simulink model "nms_sim_2D_cost"  (R2024b)
settings: Solver=ode15s  StartTime=0.0  StopTime=t_sim  MaxStep=dt_max  EnableMultiTasking=on
values from neighbouring files (symbols this model uses):
  a_BFSH = param_ctrl(35)*1    [setCtrlPar_optim_CPGreflex2001_2D.m]
  a_GAS = param_ctrl(37)*1    [setCtrlPar_optim_CPGreflex2001_2D.m]
  a_GLU = param_ctrl(31)*1    [setCtrlPar_optim_CPGreflex2001_2D.m]
  a_HAM = param_ctrl(33)*1    [setCtrlPar_optim_CPGreflex2001_2D.m]
  a_HFL = param_ctrl(32)*1    [setCtrlPar_optim_CPGreflex2001_2D.m]
  a_RF = param_ctrl(34)*1    [setCtrlPar_optim_CPGreflex2001_2D.m]
  a_SOL = param_ctrl(38)*1    [setCtrlPar_optim_CPGreflex2001_2D.m]
  a_TA = param_ctrl(39)*1    [setCtrlPar_optim_CPGreflex2001_2D.m]
  a_VAS = param_ctrl(36)*1    [setCtrlPar_optim_CPGreflex2001_2D.m]
  ai = param_ctrl(96)*2.0    [setCtrlPar_optim_CPGreflex2001_2D.m]
  b_BFSH = param_ctrl(52)*.51    [setCtrlPar_optim_CPGreflex2001_2D.m]
  b_BFSHGAS = param_ctrl(55)*.51    [setCtrlPar_optim_CPGreflex2001_2D.m]
  b_BFSHHAM = param_ctrl(54)*.51    [setCtrlPar_optim_CPGreflex2001_2D.m]
  b_BFSHVAS = param_ctrl(53)*.51    [setCtrlPar_optim_CPGreflex2001_2D.m]
  b_GAS = param_ctrl(59)*.51    [setCtrlPar_optim_CPGreflex2001_2D.m]
  b_GASBFSH = param_ctrl(60)*.51    [setCtrlPar_optim_CPGreflex2001_2D.m]
  b_GASSOL = param_ctrl(61)*.51    [setCtrlPar_optim_CPGreflex2001_2D.m]
  b_GLU = param_ctrl(40)*.51    [setCtrlPar_optim_CPGreflex2001_2D.m]
  b_GLUHAM = param_ctrl(42)*.51    [setCtrlPar_optim_CPGreflex2001_2D.m]
  b_GLUHFL = param_ctrl(41)*.51    [setCtrlPar_optim_CPGreflex2001_2D.m]
  b_HAM = param_ctrl(46)*.51    [setCtrlPar_optim_CPGreflex2001_2D.m]
  b_HAMBFSH = param_ctrl(48)*.51    [setCtrlPar_optim_CPGreflex2001_2D.m]
  b_HAMGLU = param_ctrl(47)*.51    [setCtrlPar_optim_CPGreflex2001_2D.m]
  b_HFL = param_ctrl(43)*.51    [setCtrlPar_optim_CPGreflex2001_2D.m]
  b_HFLGLU = param_ctrl(44)*.51    [setCtrlPar_optim_CPGreflex2001_2D.m]
  b_HFLRF = param_ctrl(45)*.51    [setCtrlPar_optim_CPGreflex2001_2D.m]
  b_RF = param_ctrl(49)*.51    [setCtrlPar_optim_CPGreflex2001_2D.m]
  b_RFHFL = param_ctrl(50)*.51    [setCtrlPar_optim_CPGreflex2001_2D.m]
  b_RFVAS = param_ctrl(51)*.51    [setCtrlPar_optim_CPGreflex2001_2D.m]
  b_SOL = param_ctrl(62)*.51    [setCtrlPar_optim_CPGreflex2001_2D.m]
  b_SOLGAS = param_ctrl(64)*.51    [setCtrlPar_optim_CPGreflex2001_2D.m]
  b_SOLTA = param_ctrl(63)*.51    [setCtrlPar_optim_CPGreflex2001_2D.m]
  b_TA = param_ctrl(65)*.51    [setCtrlPar_optim_CPGreflex2001_2D.m]
  b_TASOL = param_ctrl(66)*.51    [setCtrlPar_optim_CPGreflex2001_2D.m]
  b_VAS = param_ctrl(56)*.51    [setCtrlPar_optim_CPGreflex2001_2D.m]
  b_VASBFSH = param_ctrl(57)*.51    [setCtrlPar_optim_CPGreflex2001_2D.m]
  b_VASRF = param_ctrl(58)*.51    [setCtrlPar_optim_CPGreflex2001_2D.m]
  bias = param_ctrl(97)*2.5    [setCtrlPar_optim_CPGreflex2001_2D.m]
  c = 0.05    [nms_MS_2D_scaled.m]
  c_jointstop = 0.3 / (pi/180)    (= 17.1887338539)    [nms_MS_2D_scaled.m]
  D12_F = 0.16    *scaleL_JPhys    [nms_MechInit_2D_scaleSkel.m]
  D12_S = 0.2460	*sub_height    [nms_MechInit_2D_scaleSkel.m]
  D12_T = 0.2450  *sub_height    [nms_MechInit_2D_scaleSkel.m]
  D12y_F = 0.039  *sub_height    [nms_MechInit_2D_scaleSkel.m]
  D12z_HAT = 0.1    [nms_MS_2D_scaled.m]
  D13_F = 0.20    *scaleL_JPhys    [nms_MechInit_2D_scaleSkel.m]
  D1G_F = 0.14    *scaleL_JPhys    [nms_MechInit_2D_scaleSkel.m]
  D1G_HAT = 0.35  *scaleL_JPhys    [nms_MechInit_2D_scaleSkel.m]
  D1G_S = (0.3 - D12y_F/4)	*scaleL_JPhys    [nms_MechInit_2D_scaleSkel.m]
  D1G_T = (0.3 - D12y_F/4)	*scaleL_JPhys    [nms_MechInit_2D_scaleSkel.m]
  D1Gy_F = D12y_F*D1G_F/D12_F    (= 0.07)    [nms_MechInit_2D_scaleSkel.m]
  d_BFSH = param_ctrl(26)*1    [setCtrlPar_optim_CPGreflex2001_2D.m]
  d_GAS = param_ctrl(28)*1    [setCtrlPar_optim_CPGreflex2001_2D.m]
  d_GLU = param_ctrl(22)*1    [setCtrlPar_optim_CPGreflex2001_2D.m]
  d_HAM = param_ctrl(24)*1    [setCtrlPar_optim_CPGreflex2001_2D.m]
  d_HFL = param_ctrl(23)*1    [setCtrlPar_optim_CPGreflex2001_2D.m]
  d_RF = param_ctrl(25)*1    [setCtrlPar_optim_CPGreflex2001_2D.m]
  d_SOL = param_ctrl(29)*1    [setCtrlPar_optim_CPGreflex2001_2D.m]
  d_TA = param_ctrl(30)*1    [setCtrlPar_optim_CPGreflex2001_2D.m]
  d_VAS = param_ctrl(27)*1    [setCtrlPar_optim_CPGreflex2001_2D.m]
  DeltaThRef = 5e-3    (= 0.005)    [nms_MS_2D_scaled.m]
  dloptBFSH = 3.0    (= 3)    [setCtrlPar_optim_CPGreflex2001_2D.m]
  dloptGAS = 3.0    (= 3)    [setCtrlPar_optim_CPGreflex2001_2D.m]
  dloptGLU = 3.0    (= 3)    [setCtrlPar_optim_CPGreflex2001_2D.m]
  dloptHAM = 3.0    (= 3)    [setCtrlPar_optim_CPGreflex2001_2D.m]
  dloptHFL = 3.0    (= 3)    [setCtrlPar_optim_CPGreflex2001_2D.m]
  dloptRF = 3.0    (= 3)    [setCtrlPar_optim_CPGreflex2001_2D.m]
  dloptSOL = 3.0    (= 3)    [setCtrlPar_optim_CPGreflex2001_2D.m]
  dloptTA = 3.0    (= 3)    [setCtrlPar_optim_CPGreflex2001_2D.m]
  dloptVAS = 3.0    (= 3)    [setCtrlPar_optim_CPGreflex2001_2D.m]
  ec_BFSH = param_ctrl(80)*0.15    [setCtrlPar_optim_CPGreflex2001_2D.m]
  ec_GAS = param_ctrl(82)*0.15    [setCtrlPar_optim_CPGreflex2001_2D.m]
  ec_GLU = param_ctrl(76)*0.15    [setCtrlPar_optim_CPGreflex2001_2D.m]
  ec_HAM = param_ctrl(78)*0.15    [setCtrlPar_optim_CPGreflex2001_2D.m]
  ec_HFL = param_ctrl(77)*0.15    [setCtrlPar_optim_CPGreflex2001_2D.m]
  ec_RF = param_ctrl(79)*0.15    [setCtrlPar_optim_CPGreflex2001_2D.m]
  ec_TA = param_ctrl(84)*0.15    [setCtrlPar_optim_CPGreflex2001_2D.m]
  ec_VAS = param_ctrl(81)*0.15    [setCtrlPar_optim_CPGreflex2001_2D.m]
  eref = 0.04    [nms_MS_2D_scaled.m]
  eref_GAS = 0.1    [nms_MS_2D_scaled.m]
  eref_SOL = 0.1    [nms_MS_2D_scaled.m]
  es_BFSH = param_ctrl(89)*0.15    [setCtrlPar_optim_CPGreflex2001_2D.m]
  es_GAS = param_ctrl(91)*0.15    [setCtrlPar_optim_CPGreflex2001_2D.m]
  es_GLU = param_ctrl(85)*0.15    [setCtrlPar_optim_CPGreflex2001_2D.m]
  es_HAM = param_ctrl(87)*0.15    [setCtrlPar_optim_CPGreflex2001_2D.m]
  es_HFL = param_ctrl(86)*0.15    [setCtrlPar_optim_CPGreflex2001_2D.m]
  es_RF = param_ctrl(88)*0.15    [setCtrlPar_optim_CPGreflex2001_2D.m]
  es_TA = param_ctrl(93)*0.15    [setCtrlPar_optim_CPGreflex2001_2D.m]
  es_VAS = param_ctrl(90)*0.15    [setCtrlPar_optim_CPGreflex2001_2D.m]
  FmaxBFSH = 350    [nms_MS_2D_scaled.m]
  FmaxGAS = 2000    [nms_MS_2D_scaled.m]
  FmaxGLU = 4000    [nms_MS_2D_scaled.m]
  FmaxHAM = 2000    [nms_MS_2D_scaled.m]
  FmaxHFL = 2000    [nms_MS_2D_scaled.m]
  FmaxRF = 850    [nms_MS_2D_scaled.m]
  FmaxSOL = 4000    [nms_MS_2D_scaled.m]
  FmaxTA = 800    [nms_MS_2D_scaled.m]
  FmaxVAS = 5000    [nms_MS_2D_scaled.m]
  g = 9.81    [nms_MS_2D_scaled.m]
  gamma_4 = param_ctrl(11) * 1.7    [setCtrlPar_optim_CPGreflexsynergy2023_2D.m]
  h_BFSH = param_ctrl(71)*.1    [setCtrlPar_optim_CPGreflex2001_2D.m]
  h_GAS = param_ctrl(73)*.1    [setCtrlPar_optim_CPGreflex2001_2D.m]
  h_GLU = param_ctrl(67)*.1    [setCtrlPar_optim_CPGreflex2001_2D.m]
  h_HAM = param_ctrl(69)*.1    [setCtrlPar_optim_CPGreflex2001_2D.m]
  h_HFL = param_ctrl(68)*.1    [setCtrlPar_optim_CPGreflex2001_2D.m]
  h_RF = param_ctrl(70)*.1    [setCtrlPar_optim_CPGreflex2001_2D.m]
  h_SOL = param_ctrl(74)*.1    [setCtrlPar_optim_CPGreflex2001_2D.m]
  h_TA = param_ctrl(75)*.1    [setCtrlPar_optim_CPGreflex2001_2D.m]
  h_VAS = param_ctrl(72)*.1    [setCtrlPar_optim_CPGreflex2001_2D.m]
  HLCtrlPar = [theta_tgt l_clr alpha_tgt alpha_cd alpha_cv]    [setCtrlPar_optim_reflex2015_2D.m]
  In_F = 0.005    *scaleM*scaleL_JPhys^2    [nms_MechInit_2D_scaleSkel.m]
  In_HAT = 2.5    *scaleM*scaleL_JPhys^2    [nms_MechInit_2D_scaleSkel.m]
  In_S = 0.05     *scaleM*scaleL_JPhys^2    [nms_MechInit_2D_scaleSkel.m]
  In_T = 0.15     *scaleM*scaleL_JPhys^2    [nms_MechInit_2D_scaleSkel.m]
  init_exc = 0.01    [setInitPar_optim_2D.m]
  init_fm = 0.01    [setInitPar_optim_2D.m]
  init_lce = 1    [setInitPar_optim_2D.m]
  init_LCPG = param_ctrl(12) * 0.01    [setCtrlPar_optim_CPGreflexsynergy2023_2D.m]
  init_LStance = 1    [setInitPar_optim_2D.m]
  init_N1 = osc_signal1(phi_off_osc_ind)    [setCtrlPar_optim_CPGreflex2001_2D.m]
  ... (+441 more)
undefined symbols (not defined in the file or in its folder): cost_act_exponent, cost_v_tgt, flag_controller, Newton, nStep_obj, nStep_startKin, Raphson, sgn, SSW_kin, terrain_slope_angle, v_plateS1, X, Y, Z
libraries: nesl_utility x94, sm_lib x90, simulink x28, simulink_extras x12
(part 6 of 20)

== system nms_sim_2D_cost/Body Mechanics/cnt ==
  Cnt : Inport
  Cos : Trigonometry  Operator=cos
  Gain : Gain  Gain=-1
  Interpolation Using Prelookup : Interpolation_n-D  NumberOfTableDimensions=1  Table=v_plateZ  InternalRulePriority=Speed
      settings: InputPortMap=u0,u1
  Interpolation Using Prelookup1 : Interpolation_n-D  NumberOfTableDimensions=1  Table=v_plateS1  InterpMethod=Flat  InternalRulePriority=Speed
      settings: InputPortMap=u0,u1
  Mux : Mux  Inputs=5
  Prelookup : PreLookup  BreakpointsData=v_plateX  ExtrapMethod=Linear
  Selector : Selector  InputPortWidth=2  IndexOptions=Index vector (dialog)  Indices=1  OutputSizes=1
  Sin : Trigonometry
  Env : Outport
  wires:
  Cnt/1 -> Selector/1
  Prelookup/1 -> Interpolation Using Prelookup1/1, Interpolation Using Prelookup/1
  Prelookup/2 -> Interpolation Using Prelookup1/2, Interpolation Using Prelookup/2
  Selector/1 -> Prelookup/1, Mux/2
  Interpolation Using Prelookup/1 -> Mux/3, Mux/1
  Interpolation Using Prelookup1/1 -> Sin/1, Cos/1
  Sin/1 -> Gain/1
  Cos/1 -> Mux/5
  Gain/1 -> Mux/4
  Mux/1 -> Env/1

== system nms_sim_2D_cost/Body Mechanics/cnt1 ==
  Cnt : Inport
  Cos : Trigonometry  Operator=cos
  Gain : Gain  Gain=-1
  Interpolation Using Prelookup : Interpolation_n-D  NumberOfTableDimensions=1  Table=v_plateZ  InternalRulePriority=Speed
      settings: InputPortMap=u0,u1
  Interpolation Using Prelookup1 : Interpolation_n-D  NumberOfTableDimensions=1  Table=v_plateS1  InterpMethod=Flat  InternalRulePriority=Speed
      settings: InputPortMap=u0,u1
  Mux : Mux  Inputs=5
  Prelookup : PreLookup  BreakpointsData=v_plateX  ExtrapMethod=Linear
  Selector : Selector  InputPortWidth=2  IndexOptions=Index vector (dialog)  Indices=1  OutputSizes=1
  Sin : Trigonometry
  Env : Outport
  wires:
  Mux/1 -> Env/1
  Gain/1 -> Mux/4
  Cos/1 -> Mux/5
  Sin/1 -> Gain/1
  Interpolation Using Prelookup1/1 -> Cos/1, Sin/1
  Interpolation Using Prelookup/1 -> Mux/1, Mux/3
  Selector/1 -> Mux/2, Prelookup/1
  Prelookup/2 -> Interpolation Using Prelookup/2, Interpolation Using Prelookup1/2
  Prelookup/1 -> Interpolation Using Prelookup/1, Interpolation Using Prelookup1/1
  Cnt/1 -> Selector/1

== system nms_sim_2D_cost/Body Mechanics/cnt2 ==
  Cnt : Inport
  Cos : Trigonometry  Operator=cos
  Gain : Gain  Gain=-1
  Interpolation Using Prelookup : Interpolation_n-D  NumberOfTableDimensions=1  Table=v_plateZ  InternalRulePriority=Speed
      settings: InputPortMap=u0,u1
  Interpolation Using Prelookup1 : Interpolation_n-D  NumberOfTableDimensions=1  Table=v_plateS1  InterpMethod=Flat  InternalRulePriority=Speed
      settings: InputPortMap=u0,u1
  Mux : Mux  Inputs=5
  Prelookup : PreLookup  BreakpointsData=v_plateX  ExtrapMethod=Linear
  Selector : Selector  InputPortWidth=2  IndexOptions=Index vector (dialog)  Indices=1  OutputSizes=1
  Sin : Trigonometry
  Env : Outport
  wires:
  Cnt/1 -> Selector/1
  Prelookup/1 -> Interpolation Using Prelookup1/1, Interpolation Using Prelookup/1
  Prelookup/2 -> Interpolation Using Prelookup1/2, Interpolation Using Prelookup/2
  Selector/1 -> Prelookup/1, Mux/2
  Interpolation Using Prelookup/1 -> Mux/3, Mux/1
  Interpolation Using Prelookup1/1 -> Sin/1, Cos/1
  Sin/1 -> Gain/1
  Cos/1 -> Mux/5
  Gain/1 -> Mux/4
  Mux/1 -> Env/1

== system nms_sim_2D_cost/Body Mechanics/cnt3 ==
  Cnt : Inport
  Cos : Trigonometry  Operator=cos
  Gain : Gain  Gain=-1
  Interpolation Using Prelookup : Interpolation_n-D  NumberOfTableDimensions=1  Table=v_plateZ  InternalRulePriority=Speed
      settings: InputPortMap=u0,u1
  Interpolation Using Prelookup1 : Interpolation_n-D  NumberOfTableDimensions=1  Table=v_plateS1  InterpMethod=Flat  InternalRulePriority=Speed
      settings: InputPortMap=u0,u1
  Mux : Mux  Inputs=5
  Prelookup : PreLookup  BreakpointsData=v_plateX  ExtrapMethod=Linear
  Selector : Selector  InputPortWidth=2  IndexOptions=Index vector (dialog)  Indices=1  OutputSizes=1
  Sin : Trigonometry
  Env : Outport
  wires:
  Mux/1 -> Env/1
  Gain/1 -> Mux/4
  Cos/1 -> Mux/5
  Sin/1 -> Gain/1
  Interpolation Using Prelookup1/1 -> Cos/1, Sin/1
  Interpolation Using Prelookup/1 -> Mux/1, Mux/3
  Selector/1 -> Mux/2, Prelookup/1
  Prelookup/2 -> Interpolation Using Prelookup/2, Interpolation Using Prelookup1/2
  Prelookup/1 -> Interpolation Using Prelookup/1, Interpolation Using Prelookup1/1
  Cnt/1 -> Selector/1

== system nms_sim_2D_cost/Body Mechanics/contact information ==
  point : Inport
  Constant : Constant  Value=0
  Constant1 : Constant  Value=[0 0 1]
  Mux9 : Mux  Inputs=3
  Selector13 : Selector  InputPortWidth=3  IndexOptions=Index vector (dialog)  Indices=1  OutputSizes=1
  vector : Outport
  wires:
  Constant/1 -> Mux9/1
  Constant1/1 -> Mux9/3
  Mux9/1 -> vector/1
  point/1 -> Selector13/1
  Selector13/1 -> Mux9/2

== system nms_sim_2D_cost/Body Mechanics/contact information1 ==
  point : Inport
  Constant : Constant  Value=0
  Constant1 : Constant  Value=[0 0 1]
  Mux9 : Mux  Inputs=3
  Selector13 : Selector  InputPortWidth=3  IndexOptions=Index vector (dialog)  Indices=1  OutputSizes=1
  vector : Outport
  wires:
  Constant/1 -> Mux9/1
  Constant1/1 -> Mux9/3
  Mux9/1 -> vector/1
  point/1 -> Selector13/1
  Selector13/1 -> Mux9/2

== system nms_sim_2D_cost/Body Mechanics/contact information2 ==
  point : Inport
  Constant : Constant  Value=0
  Constant1 : Constant  Value=[0 0 1]
  Mux9 : Mux  Inputs=3
  Selector13 : Selector  InputPortWidth=3  IndexOptions=Index vector (dialog)  Indices=1  OutputSizes=1
  vector : Outport
  wires:
  Constant/1 -> Mux9/1
  Constant1/1 -> Mux9/3
  Mux9/1 -> vector/1
  point/1 -> Selector13/1
  Selector13/1 -> Mux9/2

== system nms_sim_2D_cost/Body Mechanics/contact information3 ==
  point : Inport
  Constant : Constant  Value=0
  Constant1 : Constant  Value=[0 0 1]
  Mux9 : Mux  Inputs=3
  Selector13 : Selector  InputPortWidth=3  IndexOptions=Index vector (dialog)  Indices=1  OutputSizes=1
  vector : Outport
  wires:
  Constant/1 -> Mux9/1
  Constant1/1 -> Mux9/3
  Mux9/1 -> vector/1
  point/1 -> Selector13/1
  Selector13/1 -> Mux9/2

== system nms_sim_2D_cost/CPG-reflex Controller/Alpha moto-neuron ==
  rhythm_ext : Inport
  GGLU : Inport  Port=2
  LMSHFL : Inport  Port=3
  LMSHAM : Inport  Port=4
  SGLU : Inport  Port=5
  Feedback : Inport  Port=6
  Constant : Constant  Value=h_GLU
  Gain1 : Gain  Gain=a_GLU
  Gain2 : Gain  Gain=1/tao_alpha
  Gain3 : Gain  Gain=d_GLU
  Gain4 : Gain  Gain=b_GLU
  Gain5 : Gain  Gain=-b_GLUHFL
  Gain6 : Gain  Gain=b_GLUHAM
  Gain7 : Gain  Gain=-1
  Integrator : Integrator  InitialCondition=init_exc
  Sum : Sum  Inputs=++++++++
  sigmoid function : Subsystem
  LExcGLU : Outport
  wires:
  Sum/1 -> Gain2/1, sigmoid function/1(u)
  SGLU/1 -> Gain4/1
  GGLU/1 -> Gain1/1
  rhythm_ext/1 -> Gain3/1
  Gain2/1 -> Integrator/1
  Integrator/1 -> Gain7/1
  Gain3/1 -> Sum/2
  Gain1/1 -> Sum/3
  Gain4/1 -> Sum/4
  Constant/1 -> Sum/8
  Feedback/1 -> Sum/7
  LMSHAM/1 -> Gain6/1
  LMSHFL/1 -> Gain5/1
  Gain5/1 -> Sum/5
  Gain6/1 -> Sum/6
  sigmoid function/1(LExcGLU) -> LExcGLU/1
  Gain7/1 -> Sum/1

== system nms_sim_2D_cost/CPG-reflex Controller/Alpha moto-neuron1 ==
  rhythm_ext : Inport
  GHAM : Inport  Port=2
  LMSGLU : Inport  Port=3
  LMSBFSH : Inport  Port=4
  SHAM : Inport  Port=5
  FBHAM : Inport  Port=6
  Constant : Constant  Value=h_HAM
  Gain1 : Gain  Gain=a_HAM
  Gain2 : Gain  Gain=1/tao_alpha
  Gain3 : Gain  Gain=d_HAM
  Gain4 : Gain  Gain=b_HAM
  Gain5 : Gain  Gain=b_HAMGLU
  Gain6 : Gain  Gain=b_HAMBFSH
  Gain7 : Gain  Gain=-1
  Integrator : Integrator  InitialCondition=init_exc
  Sum : Sum  Inputs=++++++++
  sigmoid function : Subsystem
  LExcHAM : Outport
  wires:
  Sum/1 -> Gain2/1, sigmoid function/1(u)
  SHAM/1 -> Gain4/1
  GHAM/1 -> Gain1/1
  rhythm_ext/1 -> Gain3/1
  Gain2/1 -> Integrator/1
  Integrator/1 -> Gain7/1
  Gain3/1 -> Sum/2
  Gain1/1 -> Sum/3
  Gain4/1 -> Sum/4
  Constant/1 -> Sum/8
  FBHAM/1 -> Sum/7
  LMSBFSH/1 -> Gain6/1
  LMSGLU/1 -> Gain5/1
  Gain5/1 -> Sum/5
  Gain6/1 -> Sum/6
  sigmoid function/1(LExcHAM) -> LExcHAM/1
  Gain7/1 -> Sum/1

== system nms_sim_2D_cost/CPG-reflex Controller/Alpha moto-neuron18 ==
  rhythm_ext : Inport
  GHAM : Inport  Port=2
  LMSGLU : Inport  Port=3
  LMSBFSH : Inport  Port=4
  SHAM : Inport  Port=5
  FBHAM : Inport  Port=6
  Constant : Constant  Value=h_HAM
  Gain1 : Gain  Gain=a_HAM
  Gain2 : Gain  Gain=1/tao_alpha
  Gain3 : Gain  Gain=d_HAM
  Gain4 : Gain  Gain=b_HAM
  Gain5 : Gain  Gain=b_HAMGLU
  Gain6 : Gain  Gain=b_HAMBFSH
  Gain7 : Gain  Gain=-1
  Integrator : Integrator  InitialCondition=init_exc
  Sum : Sum  Inputs=++++++++
  sigmoid function : Subsystem
  RExcHAM : Outport
  wires:
  Gain6/1 -> Sum/6
  Gain5/1 -> Sum/5
  LMSGLU/1 -> Gain5/1
  LMSBFSH/1 -> Gain6/1
  FBHAM/1 -> Sum/7
  Constant/1 -> Sum/8
  Gain4/1 -> Sum/4
  Gain1/1 -> Sum/3
  Gain3/1 -> Sum/2
  Integrator/1 -> Gain7/1
  Gain2/1 -> Integrator/1
  rhythm_ext/1 -> Gain3/1
  GHAM/1 -> Gain1/1
  SHAM/1 -> Gain4/1
  sigmoid function/1(RExc) -> RExcHAM/1
  Sum/1 -> sigmoid function/1(u), Gain2/1
  Gain7/1 -> Sum/1

== system nms_sim_2D_cost/CPG-reflex Controller/Alpha moto-neuron19 ==
  rhythm_flex : Inport
  GHFL : Inport  Port=2
  LMSGLU : Inport  Port=3
  LMSRF : Inport  Port=4
  SHFL : Inport  Port=5
  FBHFL : Inport  Port=6
  Constant : Constant  Value=h_HFL
  Gain1 : Gain  Gain=a_HFL
  Gain2 : Gain  Gain=1/tao_alpha
  Gain3 : Gain  Gain=d_HFL
  Gain4 : Gain  Gain=b_HFL
  Gain5 : Gain  Gain=-b_HFLGLU
  Gain6 : Gain  Gain=b_HFLRF
  Gain7 : Gain  Gain=-1
  Integrator : Integrator  InitialCondition=init_exc
  Scope1 : Scope
  Sum : Sum  Inputs=++++++++
  sigmoid function : Subsystem
  RExcHFL : Outport
  wires:
  Gain6/1 -> Sum/6
  Gain5/1 -> Sum/5
  LMSGLU/1 -> Gain5/1
  LMSRF/1 -> Gain6/1
  FBHFL/1 -> Sum/7
  Constant/1 -> Sum/8
  SHFL/1 -> Gain4/1
  GHFL/1 -> Gain1/1
  rhythm_flex/1 -> Gain3/1
  Gain2/1 -> Integrator/1
  Integrator/1 -> Gain7/1
  Gain3/1 -> Sum/2
  Gain1/1 -> Sum/3
  Gain4/1 -> Sum/4
  Sum/1 -> sigmoid function/1(u), Gain2/1
  sigmoid function/1(RExc) -> RExcHFL/1
  Gain7/1 -> Sum/1, Scope1/1

== system nms_sim_2D_cost/CPG-reflex Controller/Alpha moto-neuron2 ==
  rhythm_flex : Inport
  GHFL : Inport  Port=2
  LMSGLU : Inport  Port=3
  LMSRF : Inport  Port=4
  SHFL : Inport  Port=5
  FBHFL : Inport  Port=6
  Constant : Constant  Value=h_HFL
  Gain1 : Gain  Gain=a_HFL
  Gain2 : Gain  Gain=tao_alpha
  Gain3 : Gain  Gain=d_HFL
  Gain4 : Gain  Gain=b_HFL
  Gain5 : Gain  Gain=-b_HFLGLU
  Gain6 : Gain  Gain=b_HFLRF
  Gain7 : Gain  Gain=-1
  Integrator : Integrator  InitialCondition=1
  Sum : Sum  Inputs=++++++++
  sigmoid function : Subsystem
  LExcHFL : Outport
  wires:
  Gain4/1 -> Sum/4
  Gain1/1 -> Sum/3
  Gain3/1 -> Sum/2
  Integrator/1 -> Gain7/1
  Gain2/1 -> Integrator/1
  rhythm_flex/1 -> Gain3/1
  GHFL/1 -> Gain1/1
  SHFL/1 -> Gain4/1
  Constant/1 -> Sum/8
  FBHFL/1 -> Sum/7
  LMSRF/1 -> Gain6/1
  LMSGLU/1 -> Gain5/1
  Gain5/1 -> Sum/5
  Gain6/1 -> Sum/6
  Sum/1 -> sigmoid function/1(u), Gain2/1
  sigmoid function/1(LExc) -> LExcHFL/1
  Gain7/1 -> Sum/1

== system nms_sim_2D_cost/CPG-reflex Controller/Alpha moto-neuron20 ==
  rhythm_flex : Inport
  GRF : Inport  Port=2
  LMSHFL : Inport  Port=3
  LMSVAS : Inport  Port=4
  SRF : Inport  Port=5
  FBRF : Inport  Port=6
  Constant : Constant  Value=h_RF
  Gain1 : Gain  Gain=a_RF
  Gain2 : Gain  Gain=1/tao_alpha
  Gain3 : Gain  Gain=d_RF
  Gain4 : Gain  Gain=b_RF
  Gain5 : Gain  Gain=b_RFHFL
  Gain6 : Gain  Gain=b_RFVAS
  Gain7 : Gain  Gain=-1
  Integrator : Integrator  InitialCondition=init_exc
  Sum : Sum  Inputs=++++++++
  sigmoid function : Subsystem
  RExcRF : Outport
  wires:
  Gain6/1 -> Sum/6
  LMSVAS/1 -> Gain6/1
  Gain5/1 -> Sum/5
  LMSHFL/1 -> Gain5/1
  FBRF/1 -> Sum/7
  Constant/1 -> Sum/8
  SRF/1 -> Gain4/1
  GRF/1 -> Gain1/1
  rhythm_flex/1 -> Gain3/1
  Gain2/1 -> Integrator/1
  Integrator/1 -> Gain7/1
  Gain3/1 -> Sum/2
  Gain1/1 -> Sum/3
  Gain4/1 -> Sum/4
  sigmoid function/1(RExc) -> RExcRF/1
  Sum/1 -> sigmoid function/1(u), Gain2/1
  Gain7/1 -> Sum/1

== system nms_sim_2D_cost/CPG-reflex Controller/Alpha moto-neuron21 ==
  rhythm_ext : Inport
  GBFSH : Inport  Port=2
  LMSVAS : Inport  Port=3
  LMSGAS : Inport  Port=4
  LMSHAM : Inport  Port=5
  SBFSH : Inport  Port=6
  FBBFSH : Inport  Port=7
  Constant : Constant  Value=h_BFSH
  Gain1 : Gain  Gain=a_BFSH
  Gain2 : Gain  Gain=1/tao_alpha
  Gain3 : Gain  Gain=d_BFSH
  Gain4 : Gain  Gain=b_BFSH
  Gain5 : Gain  Gain=-b_BFSHVAS
  Gain6 : Gain  Gain=b_BFSHGAS
  Gain7 : Gain  Gain=b_BFSHHAM
  Gain8 : Gain  Gain=-1
  Integrator : Integrator  InitialCondition=init_exc
  Sum : Sum  Inputs=+++++++++
  sigmoid function : Subsystem
  RExcBFSH : Outport
  wires:
  Gain7/1 -> Sum/7
  Gain6/1 -> Sum/6
  Gain5/1 -> Sum/5
  LMSVAS/1 -> Gain5/1
  LMSGAS/1 -> Gain6/1
  LMSHAM/1 -> Gain7/1
  FBBFSH/1 -> Sum/8
  Constant/1 -> Sum/9
  SBFSH/1 -> Gain4/1
  GBFSH/1 -> Gain1/1
  rhythm_ext/1 -> Gain3/1
  Gain2/1 -> Integrator/1
  Integrator/1 -> Gain8/1
  Gain3/1 -> Sum/2
  Gain1/1 -> Sum/3
  Gain4/1 -> Sum/4
  Sum/1 -> sigmoid function/1(u), Gain2/1
  sigmoid function/1(RExc) -> RExcBFSH/1
  Gain8/1 -> Sum/1

== system nms_sim_2D_cost/CPG-reflex Controller/Alpha moto-neuron22 ==
  rhythm_flex : Inport
  GVAS : Inport  Port=2
  LMSBFSH : Inport  Port=3
  LMSRF : Inport  Port=4
  SVAS : Inport  Port=5
  FBVAS : Inport  Port=6
  Constant : Constant  Value=h_VAS
  Gain1 : Gain  Gain=a_VAS
  Gain2 : Gain  Gain=1/tao_alpha
  Gain3 : Gain  Gain=d_VAS
  Gain4 : Gain  Gain=b_VAS
  Gain5 : Gain  Gain=b_VASRF
  Gain6 : Gain  Gain=-b_VASBFSH
  Gain7 : Gain  Gain=-1
  Integrator : Integrator  InitialCondition=init_exc
  Sum : Sum  Inputs=++++++++
  sigmoid function : Subsystem
  RExcVAS : Outport
  wires:
  Gain6/1 -> Sum/5  "msbfsh"
  Gain5/1 -> Sum/6  "msrf"
  LMSRF/1 -> Gain5/1
  LMSBFSH/1 -> Gain6/1
  FBVAS/1 -> Sum/7  "fb"
  Constant/1 -> Sum/8  "h"
  Gain4/1 -> Sum/4  "ms"
  Gain1/1 -> Sum/3  "golgi"
  Gain3/1 -> Sum/2  "rhythm"
  Integrator/1 -> Gain7/1  "aloha"
  Gain2/1 -> Integrator/1
  rhythm_flex/1 -> Gain3/1
  GVAS/1 -> Gain1/1
  SVAS/1 -> Gain4/1
  Sum/1 -> sigmoid function/1(u), Gain2/1
  sigmoid function/1(RExc) -> RExcVAS/1
  Gain7/1 -> Sum/1

== system nms_sim_2D_cost/CPG-reflex Controller/Alpha moto-neuron23 ==
  rhythm_ext : Inport
  GSOL : Inport  Port=2
  LMSTA : Inport  Port=3
  LMSGAS : Inport  Port=4
  SSOL : Inport  Port=5
  FB SOL : Inport  Port=6
  Constant : Constant  Value=h_SOL
  Gain1 : Gain  Gain=a_SOL
  Gain2 : Gain  Gain=1/tao_alpha
  Gain3 : Gain  Gain=d_SOL
  Gain4 : Gain  Gain=b_SOL
  Gain5 : Gain  Gain=-b_SOLTA
  Gain6 : Gain  Gain=b_SOLGAS
  Gain7 : Gain  Gain=-1
  Integrator : Integrator  InitialCondition=init_exc
  Sum : Sum  Inputs=++++++++
  sigmoid function : Subsystem
  RExcSOL : Outport
  wires:
  Gain6/1 -> Sum/6
  Gain5/1 -> Sum/5
  LMSTA/1 -> Gain5/1
  LMSGAS/1 -> Gain6/1
  FB SOL/1 -> Sum/7
  Constant/1 -> Sum/8
  Gain4/1 -> Sum/4
  Gain1/1 -> Sum/3
  Gain3/1 -> Sum/2
  Integrator/1 -> Gain7/1
  Gain2/1 -> Integrator/1
  rhythm_ext/1 -> Gain3/1
  GSOL/1 -> Gain1/1
  SSOL/1 -> Gain4/1
  sigmoid function/1(RExc) -> RExcSOL/1
  Sum/1 -> sigmoid function/1(u), Gain2/1
  Gain7/1 -> Sum/1

== system nms_sim_2D_cost/CPG-reflex Controller/Alpha moto-neuron24 ==
  rhythm_flex : Inport
  GTA : Inport  Port=2
  LMSSOL : Inport  Port=3
  STA : Inport  Port=4
  FB TA : Inport  Port=5
  Constant : Constant  Value=h_TA
  Gain1 : Gain  Gain=a_TA
  Gain2 : Gain  Gain=1/tao_alpha
  Gain3 : Gain  Gain=d_TA
  Gain4 : Gain  Gain=b_TA
  Gain5 : Gain  Gain=-b_TASOL
  Gain7 : Gain  Gain=-1
  Integrator : Integrator  InitialCondition=init_exc
  Sum : Sum  Inputs=+++++++
  sigmoid function : Subsystem
  RExcTA : Outport
  wires:
  FB TA/1 -> Sum/6
  Gain5/1 -> Sum/5
  LMSSOL/1 -> Gain5/1
  Constant/1 -> Sum/7
  STA/1 -> Gain4/1
  GTA/1 -> Gain1/1
  rhythm_flex/1 -> Gain3/1
  Gain2/1 -> Integrator/1
  Integrator/1 -> Gain7/1
  Gain3/1 -> Sum/2
  Gain1/1 -> Sum/3
  Gain4/1 -> Sum/4
  Sum/1 -> sigmoid function/1(u), Gain2/1
  Gain7/1 -> Sum/1
  sigmoid function/1(RExc) -> RExcTA/1

== system nms_sim_2D_cost/CPG-reflex Controller/Alpha moto-neuron25 ==
  rhythm_ext : Inport
  GGAS : Inport  Port=2
  LMSBFSH : Inport  Port=3
  LMSSOL : Inport  Port=4
  SGAS : Inport  Port=5
  FBGAS : Inport  Port=6
  Constant : Constant  Value=h_GAS
  Gain1 : Gain  Gain=a_GAS
  Gain2 : Gain  Gain=1/tao_alpha
  Gain3 : Gain  Gain=d_GAS
  Gain4 : Gain  Gain=b_GAS
  Gain5 : Gain  Gain=b_GASBFSH
  Gain6 : Gain  Gain=b_GASSOL
  Gain7 : Gain  Gain=-1
  Integrator : Integrator  InitialCondition=init_exc
  Sum : Sum  Inputs=++++++++
  sigmoid function : Subsystem
  RExcGAS : Outport
  wires:
  Gain6/1 -> Sum/6
  Gain5/1 -> Sum/5
  LMSBFSH/1 -> Gain5/1
  LMSSOL/1 -> Gain6/1
  FBGAS/1 -> Sum/7
  Constant/1 -> Sum/8
  SGAS/1 -> Gain4/1
  GGAS/1 -> Gain1/1
  rhythm_ext/1 -> Gain3/1
  Gain2/1 -> Integrator/1
  Integrator/1 -> Gain7/1
  Gain3/1 -> Sum/2
  Gain1/1 -> Sum/3
  Gain4/1 -> Sum/4
  Sum/1 -> sigmoid function/1(u), Gain2/1
  sigmoid function/1(RExc) -> RExcGAS/1
  Gain7/1 -> Sum/1

== system nms_sim_2D_cost/CPG-reflex Controller/Alpha moto-neuron26 ==
  rhythm_ext : Inport
  GGLU : Inport  Port=2
  LMSHFL : Inport  Port=3
  LMSHAM : Inport  Port=4
  SGLU : Inport  Port=5
  Feedback : Inport  Port=6
  Constant : Constant  Value=h_GLU
  Gain1 : Gain  Gain=a_GLU
  Gain2 : Gain  Gain=1/tao_alpha
  Gain3 : Gain  Gain=d_GLU
  Gain4 : Gain  Gain=b_GLU
  Gain5 : Gain  Gain=-b_GLUHFL
  Gain6 : Gain  Gain=b_GLUHAM
  Gain7 : Gain  Gain=-1
  Integrator : Integrator  InitialCondition=init_exc
  Sum : Sum  Inputs=++++++++
  sigmoid function : Subsystem
  RExcGLU : Outport
  wires:
  Gain6/1 -> Sum/6
  Gain5/1 -> Sum/5
  LMSHFL/1 -> Gain5/1
  LMSHAM/1 -> Gain6/1
  Feedback/1 -> Sum/7
  Constant/1 -> Sum/8
  Gain4/1 -> Sum/4
  Gain1/1 -> Sum/3
  Gain3/1 -> Sum/2
  Integrator/1 -> Gain7/1
  Gain2/1 -> Integrator/1
  rhythm_ext/1 -> Gain3/1
  GGLU/1 -> Gain1/1
  SGLU/1 -> Gain4/1
  sigmoid function/1(RExc) -> RExcGLU/1
  Sum/1 -> Gain2/1, sigmoid function/1(u)
  Gain7/1 -> Sum/1

== system nms_sim_2D_cost/CPG-reflex Controller/Alpha moto-neuron3 ==
  rhythm_flex : Inport
  GRF : Inport  Port=2
  LMSHFL : Inport  Port=3
  LMSVAS : Inport  Port=4
  SRF : Inport  Port=5
  FBRF : Inport  Port=6
  Constant : Constant  Value=h_RF
  Gain1 : Gain  Gain=a_RF
  Gain2 : Gain  Gain=1/tao_alpha
  Gain3 : Gain  Gain=d_RF
  Gain4 : Gain  Gain=b_RF
  Gain5 : Gain  Gain=b_RFHFL
  Gain6 : Gain  Gain=b_RFVAS
  Gain7 : Gain  Gain=-1
  Integrator : Integrator  InitialCondition=init_exc
  Sum : Sum  Inputs=++++++++
  sigmoid function : Subsystem
  LExcRF : Outport
  wires:
  Gain4/1 -> Sum/4
  Gain1/1 -> Sum/3
  Gain3/1 -> Sum/2
  Integrator/1 -> Gain7/1
  Gain2/1 -> Integrator/1
  rhythm_flex/1 -> Gain3/1
  GRF/1 -> Gain1/1
  SRF/1 -> Gain4/1
  Constant/1 -> Sum/8
  FBRF/1 -> Sum/7
  LMSHFL/1 -> Gain5/1
  Gain5/1 -> Sum/5
  LMSVAS/1 -> Gain6/1
  Gain6/1 -> Sum/6
  Sum/1 -> sigmoid function/1(u), Gain2/1
  sigmoid function/1(LExc) -> LExcRF/1
  Gain7/1 -> Sum/1

== system nms_sim_2D_cost/CPG-reflex Controller/Alpha moto-neuron4 ==
  rhythm_ext : Inport
  GBFSH : Inport  Port=2
  LMSVAS : Inport  Port=3
  LMSGAS : Inport  Port=4
  LMSHAM : Inport  Port=5
  SBFSH : Inport  Port=6
  FBBFSH : Inport  Port=7
  Constant : Constant  Value=h_BFSH
  Gain1 : Gain  Gain=a_BFSH
  Gain2 : Gain  Gain=1/tao_alpha
  Gain3 : Gain  Gain=d_BFSH
  Gain4 : Gain  Gain=b_BFSH
  Gain5 : Gain  Gain=-b_BFSHVAS
  Gain6 : Gain  Gain=b_BFSHGAS
  Gain7 : Gain  Gain=b_BFSHHAM
  Gain8 : Gain  Gain=-1
  Integrator : Integrator  InitialCondition=init_exc
  Sum : Sum  Inputs=+++++++++
  sigmoid function : Subsystem
  LExcBFSH : Outport
  wires:
  Gain4/1 -> Sum/4
  Gain1/1 -> Sum/3
  Gain3/1 -> Sum/2
  Integrator/1 -> Gain8/1
  Gain2/1 -> Integrator/1
  rhythm_ext/1 -> Gain3/1
  GBFSH/1 -> Gain1/1
  SBFSH/1 -> Gain4/1
  Constant/1 -> Sum/9
  FBBFSH/1 -> Sum/8
  LMSHAM/1 -> Gain7/1
  LMSGAS/1 -> Gain6/1
  LMSVAS/1 -> Gain5/1
  Gain5/1 -> Sum/5
  Gain6/1 -> Sum/6
  Gain7/1 -> Sum/7
  Sum/1 -> sigmoid function/1(u), Gain2/1
  sigmoid function/1(LExcBFSH) -> LExcBFSH/1
  Gain8/1 -> Sum/1

== system nms_sim_2D_cost/CPG-reflex Controller/Alpha moto-neuron5 ==
  rhythm_flex : Inport
  GVAS : Inport  Port=2
  LMSBFSH : Inport  Port=3
  LMSRF : Inport  Port=4
  SVAS : Inport  Port=5
  FBVAS : Inport  Port=6
  Constant : Constant  Value=h_VAS
  Gain1 : Gain  Gain=a_VAS
  Gain2 : Gain  Gain=1/tao_alpha
  Gain3 : Gain  Gain=d_VAS
  Gain4 : Gain  Gain=b_VAS
  Gain5 : Gain  Gain=b_VASRF
  Gain6 : Gain  Gain=-b_VASBFSH
  Gain7 : Gain  Gain=-1
  Integrator : Integrator  InitialCondition=init_exc
  Sum : Sum  Inputs=++++++++
  sigmoid function : Subsystem
  LExcVAS : Outport
  wires:
  SVAS/1 -> Gain4/1
  GVAS/1 -> Gain1/1
  rhythm_flex/1 -> Gain3/1
  Gain2/1 -> Integrator/1
  Integrator/1 -> Gain7/1
  Gain3/1 -> Sum/2
  Gain1/1 -> Sum/3
  Gain4/1 -> Sum/4
  Constant/1 -> Sum/8
  FBVAS/1 -> Sum/7
  LMSBFSH/1 -> Gain6/1
  LMSRF/1 -> Gain5/1
  Gain5/1 -> Sum/6
  Gain6/1 -> Sum/5
  Sum/1 -> sigmoid function/1(u), Gain2/1
  Gain7/1 -> Sum/1
  sigmoid function/1(LExc) -> LExcVAS/1

== system nms_sim_2D_cost/CPG-reflex Controller/Alpha moto-neuron6 ==
  rhythm_ext : Inport
  GSOL : Inport  Port=2
  LMSTA : Inport  Port=3
  LMSGAS : Inport  Port=4
  SSOL : Inport  Port=5
  FB SOL : Inport  Port=6
  Constant : Constant  Value=h_SOL
  Gain1 : Gain  Gain=a_SOL
  Gain2 : Gain  Gain=1/tao_alpha
  Gain3 : Gain  Gain=d_SOL
  Gain4 : Gain  Gain=b_SOL
  Gain5 : Gain  Gain=-b_SOLTA
  Gain6 : Gain  Gain=b_SOLGAS
  Gain7 : Gain  Gain=-1
  Integrator : Integrator  InitialCondition=init_exc
  Sum : Sum  Inputs=++++++++
  sigmoid function : Subsystem
  LExcSOL : Outport
  wires:
  SSOL/1 -> Gain4/1
  GSOL/1 -> Gain1/1
  rhythm_ext/1 -> Gain3/1
  Gain2/1 -> Integrator/1
  Integrator/1 -> Gain7/1  "alpha"
  Gain3/1 -> Sum/2  "rhythm"
  Gain1/1 -> Sum/3  "golgi"
  Gain4/1 -> Sum/4  "ms"
  Constant/1 -> Sum/8  "h"
  FB SOL/1 -> Sum/7  "fb"
  LMSGAS/1 -> Gain6/1
  LMSTA/1 -> Gain5/1
  Gain5/1 -> Sum/5  "msta"
  Gain6/1 -> Sum/6  "msgas"
  sigmoid function/1(LExcSOL) -> LExcSOL/1
  Sum/1 -> sigmoid function/1(u), Gain2/1
  Gain7/1 -> Sum/1

== system nms_sim_2D_cost/CPG-reflex Controller/Alpha moto-neuron7 ==
  rhythm_flex : Inport
  GTA : Inport  Port=2
  LMSSOL : Inport  Port=3
  STA : Inport  Port=4
  FB TA : Inport  Port=5
  Constant : Constant  Value=h_TA
  Gain1 : Gain  Gain=a_TA
  Gain2 : Gain  Gain=1/tao_alpha
  Gain3 : Gain  Gain=d_TA
  Gain4 : Gain  Gain=b_TA
  Gain5 : Gain  Gain=-b_TASOL
  Gain7 : Gain  Gain=-1
  Integrator : Integrator  InitialCondition=init_exc
  Sum : Sum  Inputs=+++++++
  sigmoid function : Subsystem
  LExcTA : Outport
  wires:
  Gain4/1 -> Sum/4
  Gain1/1 -> Sum/3
  Gain3/1 -> Sum/2
  Integrator/1 -> Gain7/1
  Gain2/1 -> Integrator/1
  rhythm_flex/1 -> Gain3/1
  GTA/1 -> Gain1/1
  STA/1 -> Gain4/1
  Constant/1 -> Sum/7
  LMSSOL/1 -> Gain5/1
  Gain5/1 -> Sum/5
  FB TA/1 -> Sum/6
  sigmoid function/1(LExcTA) -> LExcTA/1
  Sum/1 -> sigmoid function/1(u), Gain2/1
  Gain7/1 -> Sum/1

== system nms_sim_2D_cost/CPG-reflex Controller/Alpha moto-neuron8 ==
  rhythm_ext : Inport
  GGAS : Inport  Port=2
  LMSBFSH : Inport  Port=3
  LMSSOL : Inport  Port=4
  SGAS : Inport  Port=5
  FBGAS : Inport  Port=6
  Constant : Constant  Value=h_GAS
  Gain1 : Gain  Gain=a_GAS
  Gain2 : Gain  Gain=1/tao_alpha
  Gain3 : Gain  Gain=d_GAS
  Gain4 : Gain  Gain=b_GAS
  Gain5 : Gain  Gain=b_GASBFSH
  Gain6 : Gain  Gain=b_GASSOL
  Gain7 : Gain  Gain=-1
  Integrator : Integrator  InitialCondition=init_exc
  Sum : Sum  Inputs=++++++++
  sigmoid function : Subsystem
  LExcGAS : Outport
  wires:
  Gain4/1 -> Sum/4
  Gain1/1 -> Sum/3
  Gain3/1 -> Sum/2
  Integrator/1 -> Gain7/1
  Gain2/1 -> Integrator/1
  rhythm_ext/1 -> Gain3/1
  GGAS/1 -> Gain1/1
  SGAS/1 -> Gain4/1
  Constant/1 -> Sum/8
  FBGAS/1 -> Sum/7
  LMSSOL/1 -> Gain6/1
  LMSBFSH/1 -> Gain5/1
  Gain5/1 -> Sum/5
  Gain6/1 -> Sum/6
  sigmoid function/1(LExcBFSH) -> LExcGAS/1
  Sum/1 -> sigmoid function/1(u), Gain2/1
  Gain7/1 -> Sum/1

== system nms_sim_2D_cost/CPG-reflex Controller/CPG ==
  note: Adaptation
  note: Adaptation
  note: External stimulation
  note: Neuron 1
  note: Neuron 2
  FB : Inport
  Constant5 : Constant  Value=s_ext
  Gain1 : Gain  Gain=1/tao_r
  Gain10 : Gain  Gain=-1
  Gain11 : Gain  Gain=1/tao_a
  Gain14 : Gain  Gain=-1
  Gain15 : Gain  Gain=1/tao_a
  Gain16 : Gain  Gain=ai
  Gain17 : Gain  Gain=bias
  Gain18 : Gain  Gain=ai
  Gain2 : Gain  Gain=bias
  Gain3 : Gain  Gain=1/tao_r
  Integrator4 : Integrator  InitialCondition=init_N1
  Integrator5 : Integrator  InitialCondition=init_V1
  Integrator6 : Integrator  InitialCondition=init_N2
  Integrator7 : Integrator  InitialCondition=init_V2
  Max2 : MinMax  Function=max  Inputs=2
  Max3 : MinMax  Function=max  Inputs=2
  Sum4 : Sum  Inputs=--+-+
  Sum5 : Sum
  Sum6 : Sum  Inputs=--+-+
  Sum7 : Sum
  Zero : Constant  Value=0  OutDataTypeStr=Inherit: Inherit via back propagation
  Zero1 : Constant  Value=0  OutDataTypeStr=Inherit: Inherit via back propagation
  Outport : Outport
  Outport1 : Outport  Port=2
  wires:
  FB/1 -> Sum6/5, Sum4/5
  Sum5/1 -> Gain11/1
  Gain3/1 -> Integrator6/1
  Zero1/1 -> Max3/2
  Constant5/1 -> [s]
  Gain11/1 -> Integrator5/1
  Gain16/1 -> Sum6/4  "-a*max(x2, 0)"
  Zero/1 -> Max2/2
  Gain18/1 -> Sum4/4  "-a*max(x2, 0)"
  Integrator4/1 -> Max2/1, Sum4/1  "x"
  Max2/1 -> Sum5/2, Gain16/1, Outport/1
  Sum6/1 -> Gain3/1
  Gain10/1 -> Sum5/1  "-f"
  Sum4/1 -> Gain1/1
  Gain14/1 -> Sum7/1  "-f"
  Integrator7/1 -> Gain17/1, Gain14/1  "f"
  Integrator6/1 -> Sum6/1, Max3/1  "x"
  Max3/1 -> Sum7/2, Outport1/1, Gain18/1
  Gain2/1 -> Sum4/2  "bf"
  Gain1/1 -> Integrator4/1
  [s] -> Sum6/3  "s"
  Gain17/1 -> Sum6/2  "bf"
  [s] -> Sum4/3  "s"
  Gain15/1 -> Integrator7/1
  Sum7/1 -> Gain15/1
  Integrator5/1 -> Gain10/1, Gain2/1  "f"

== system nms_sim_2D_cost/CPG-reflex Controller/FB VAS ==
  LStance : Inport
  Constant : Constant
  Gain : Gain  Gain=ec_VAS
  Gain1 : Gain  Gain=es_VAS
  Sum : Sum  Inputs=|-+
  Sum1 : Sum  Inputs=|++
  FBVAS : Outport
  wires:
  LStance/1 -> Sum/1, Gain/1
  Constant/1 -> Sum/2
  Gain/1 -> Sum1/1
  Sum1/1 -> FBVAS/1
  Sum/1 -> Gain1/1
  Gain1/1 -> Sum1/2

== system nms_sim_2D_cost/CPG-reflex Controller/FB VAS2 ==
  RStance : Inport
  Constant : Constant
  Gain : Gain  Gain=ec_VAS
  Gain1 : Gain  Gain=es_VAS
  Sum : Sum  Inputs=|-+
  Sum1 : Sum  Inputs=|++
  FBVAS : Outport
  wires:
  Gain1/1 -> Sum1/2
  Sum/1 -> Gain1/1
  Sum1/1 -> FBVAS/1
  Gain/1 -> Sum1/1
  Constant/1 -> Sum/2
  RStance/1 -> Gain/1, Sum/1

== system nms_sim_2D_cost/CPG-reflex Controller/Feedback HAM ==
  LStance : Inport
  Constant : Constant
  Gain : Gain  Gain=ec_HAM
  Gain1 : Gain  Gain=es_HAM
  Sum : Sum  Inputs=|-+
  Sum1 : Sum  Inputs=|++
  FBHAM : Outport
  wires:
  LStance/1 -> Sum/1, Gain/1
  Constant/1 -> Sum/2
  Gain/1 -> Sum1/1
  Sum1/1 -> FBHAM/1
  Sum/1 -> Gain1/1
  Gain1/1 -> Sum1/2

== system nms_sim_2D_cost/CPG-reflex Controller/Feedback HAM2 ==
  RStance : Inport
  Constant : Constant
  Gain : Gain  Gain=ec_HAM
  Gain1 : Gain  Gain=es_HAM
  Sum : Sum  Inputs=|-+
  Sum1 : Sum  Inputs=|++
  FBHAM : Outport
  wires:
  Gain1/1 -> Sum1/2
  Sum/1 -> Gain1/1
  Sum1/1 -> FBHAM/1
  Gain/1 -> Sum1/1
  Constant/1 -> Sum/2
  RStance/1 -> Gain/1, Sum/1

== system nms_sim_2D_cost/CPG-reflex Controller/Golgi tendon organ BFSH ==
  FBFSH : Inport
  Gain : Gain  Gain=-1
  Gain1 : Gain  Gain=1/tao_golgi
  Integrator : Integrator  InitialCondition=init_fm
  Max : MinMax  Function=max  Inputs=2
  Sum : Sum
  Zero : Constant  Value=0  OutDataTypeStr=Inherit: Inherit via back propagation
  GBFSH : Outport
  wires:
  Gain1/1 -> Integrator/1
  Sum/1 -> Max/1, Gain1/1
  FBFSH/1 -> Sum/2
  Gain/1 -> Sum/1
  Integrator/1 -> Gain/1
  Zero/1 -> Max/2
  Max/1 -> GBFSH/1

== system nms_sim_2D_cost/CPG-reflex Controller/Golgi tendon organ BFSH2 ==
  FBFSH : Inport
  Gain : Gain  Gain=-1
  Gain1 : Gain  Gain=1/tao_golgi
  Integrator : Integrator  InitialCondition=init_fm
  Max : MinMax  Function=max  Inputs=2
  Sum : Sum
  Zero : Constant  Value=0  OutDataTypeStr=Inherit: Inherit via back propagation
  GBFSH : Outport
  wires:
  Max/1 -> GBFSH/1
  Zero/1 -> Max/2
  Integrator/1 -> Gain/1
  Gain/1 -> Sum/1
  FBFSH/1 -> Sum/2
  Sum/1 -> Gain1/1, Max/1
  Gain1/1 -> Integrator/1

== system nms_sim_2D_cost/CPG-reflex Controller/Golgi tendon organ GAS ==
  FmGAS : Inport
  Gain : Gain  Gain=-1
  Gain1 : Gain  Gain=1/tao_golgi
  Integrator : Integrator  InitialCondition=init_fm
  Max : MinMax  Function=max  Inputs=2
  Sum : Sum
  Zero : Constant  Value=0  OutDataTypeStr=Inherit: Inherit via back propagation
  GGAS : Outport
  wires:
  Gain1/1 -> Integrator/1
  Sum/1 -> Max/1, Gain1/1
  FmGAS/1 -> Sum/2
  Gain/1 -> Sum/1
  Integrator/1 -> Gain/1
  Zero/1 -> Max/2
  Max/1 -> GGAS/1

== system nms_sim_2D_cost/CPG-reflex Controller/Golgi tendon organ GAS2 ==
  FmGAS : Inport
  Gain : Gain  Gain=-1
  Gain1 : Gain  Gain=1/tao_golgi
  Integrator : Integrator  InitialCondition=init_fm
  Max : MinMax  Function=max  Inputs=2
  Sum : Sum
  Zero : Constant  Value=0  OutDataTypeStr=Inherit: Inherit via back propagation
  GGAS : Outport
  wires:
  Max/1 -> GGAS/1
  Zero/1 -> Max/2
  Integrator/1 -> Gain/1
  Gain/1 -> Sum/1
  FmGAS/1 -> Sum/2
  Sum/1 -> Gain1/1, Max/1
  Gain1/1 -> Integrator/1

== system nms_sim_2D_cost/CPG-reflex Controller/Golgi tendon organ GLU ==
  Fm : Inport
  Gain : Gain  Gain=-1
  Gain1 : Gain  Gain=1/tao_golgi
  Integrator : Integrator  InitialCondition=init_fm
  Max : MinMax  Function=max  Inputs=2
  Sum : Sum
  Zero : Constant  Value=0  OutDataTypeStr=Inherit: Inherit via back propagation
  Gm : Outport
  wires:
  Max/1 -> Gm/1
  Zero/1 -> Max/2
  Integrator/1 -> Gain/1
  Gain/1 -> Sum/1
  Fm/1 -> Sum/2
  Sum/1 -> Gain1/1, Max/1
  Gain1/1 -> Integrator/1

== system nms_sim_2D_cost/CPG-reflex Controller/Golgi tendon organ GLU2 ==
  Fm : Inport
  Gain : Gain  Gain=-1
  Gain1 : Gain  Gain=1/tao_golgi
  Integrator : Integrator  InitialCondition=init_fm
  Max : MinMax  Function=max  Inputs=2
  Sum : Sum
  Zero : Constant  Value=0  OutDataTypeStr=Inherit: Inherit via back propagation
  GGLU : Outport
  wires:
  Gain1/1 -> Integrator/1
  Sum/1 -> Max/1, Gain1/1
  Fm/1 -> Sum/2
  Gain/1 -> Sum/1
  Integrator/1 -> Gain/1
  Zero/1 -> Max/2
  Max/1 -> GGLU/1

== system nms_sim_2D_cost/CPG-reflex Controller/Golgi tendon organ HAM ==
  Fm : Inport
  Gain : Gain  Gain=-1
  Gain1 : Gain  Gain=1/tao_golgi
  Integrator : Integrator  InitialCondition=init_fm
  Max : MinMax  Function=max  Inputs=2
  Sum : Sum
  Zero : Constant  Value=0  OutDataTypeStr=Inherit: Inherit via back propagation
  Gm : Outport
  wires:
  Max/1 -> Gm/1
  Zero/1 -> Max/2
  Integrator/1 -> Gain/1
  Gain/1 -> Sum/1
  Fm/1 -> Sum/2
  Sum/1 -> Gain1/1, Max/1
  Gain1/1 -> Integrator/1

== system nms_sim_2D_cost/CPG-reflex Controller/Golgi tendon organ HAM2 ==
  FHAM : Inport
  Gain : Gain  Gain=-1
  Gain1 : Gain  Gain=1/tao_golgi
  Integrator : Integrator  InitialCondition=init_fm
  Max : MinMax  Function=max  Inputs=2
  Sum : Sum
  Zero : Constant  Value=0  OutDataTypeStr=Inherit: Inherit via back propagation
  GHAM : Outport
  wires:
  Gain1/1 -> Integrator/1
  Sum/1 -> Max/1, Gain1/1
  FHAM/1 -> Sum/2
  Gain/1 -> Sum/1
  Integrator/1 -> Gain/1
  Zero/1 -> Max/2
  Max/1 -> GHAM/1

== system nms_sim_2D_cost/CPG-reflex Controller/Golgi tendon organ HFL ==
  FmHFL : Inport
  Gain : Gain  Gain=-1
  Gain1 : Gain  Gain=1/tao_golgi
  Integrator : Integrator  InitialCondition=init_fm
  Max : MinMax  Function=max  Inputs=2
  Sum : Sum
  Zero : Constant  Value=0  OutDataTypeStr=Inherit: Inherit via back propagation
  GHFL : Outport
  wires:
  Gain1/1 -> Integrator/1
  Sum/1 -> Max/1, Gain1/1
  FmHFL/1 -> Sum/2
  Gain/1 -> Sum/1
  Integrator/1 -> Gain/1
  Zero/1 -> Max/2
  Max/1 -> GHFL/1

== system nms_sim_2D_cost/CPG-reflex Controller/Golgi tendon organ HFL2 ==
  FmHFL : Inport
  Gain : Gain  Gain=-1
  Gain1 : Gain  Gain=1/tao_golgi
  Integrator : Integrator  InitialCondition=init_fm
  Max : MinMax  Function=max  Inputs=2
  Sum : Sum
  Zero : Constant  Value=0  OutDataTypeStr=Inherit: Inherit via back propagation
  GHFL : Outport
  wires:
  Max/1 -> GHFL/1
  Zero/1 -> Max/2
  Integrator/1 -> Gain/1
  Gain/1 -> Sum/1
  FmHFL/1 -> Sum/2
  Sum/1 -> Gain1/1, Max/1
  Gain1/1 -> Integrator/1

== system nms_sim_2D_cost/CPG-reflex Controller/Golgi tendon organ RF ==
  FRF : Inport
  Gain : Gain  Gain=-1
  Gain1 : Gain  Gain=1/tao_golgi
  Integrator : Integrator  InitialCondition=init_fm
  Max : MinMax  Function=max  Inputs=2
  Sum : Sum
  Zero : Constant  Value=0  OutDataTypeStr=Inherit: Inherit via back propagation
  GRF : Outport
  wires:
  Gain1/1 -> Integrator/1
  Sum/1 -> Max/1, Gain1/1
  FRF/1 -> Sum/2
  Gain/1 -> Sum/1
  Integrator/1 -> Gain/1
  Zero/1 -> Max/2
  Max/1 -> GRF/1

== system nms_sim_2D_cost/CPG-reflex Controller/Golgi tendon organ RF2 ==
  FRF : Inport
  Gain : Gain  Gain=-1
  Gain1 : Gain  Gain=1/tao_golgi
  Integrator : Integrator  InitialCondition=init_fm
  Max : MinMax  Function=max  Inputs=2
  Sum : Sum
  Zero : Constant  Value=0  OutDataTypeStr=Inherit: Inherit via back propagation
  GRF : Outport
  wires:
  Max/1 -> GRF/1
  Zero/1 -> Max/2
  Integrator/1 -> Gain/1
  Gain/1 -> Sum/1
  FRF/1 -> Sum/2
  Sum/1 -> Gain1/1, Max/1
  Gain1/1 -> Integrator/1

== system nms_sim_2D_cost/CPG-reflex Controller/Golgi tendon organ SOL ==
  FmSOL : Inport
  Gain : Gain  Gain=-1
  Gain1 : Gain  Gain=1/tao_golgi
  Integrator : Integrator  InitialCondition=init_fm
  Max : MinMax  Function=max  Inputs=2
  Sum : Sum
  Zero : Constant  Value=0  OutDataTypeStr=Inherit: Inherit via back propagation
  GSOL : Outport
  wires:
  Max/1 -> GSOL/1
  Zero/1 -> Max/2
  Integrator/1 -> Gain/1
  Gain/1 -> Sum/1
  FmSOL/1 -> Sum/2
  Sum/1 -> Gain1/1, Max/1
  Gain1/1 -> Integrator/1

== system nms_sim_2D_cost/CPG-reflex Controller/Golgi tendon organ SOL2 ==
  FmSOL : Inport
  Gain : Gain  Gain=-1
  Gain1 : Gain  Gain=1/tao_golgi
  Integrator : Integrator  InitialCondition=init_fm
  Max : MinMax  Function=max  Inputs=2
  Sum : Sum
  Zero : Constant  Value=0  OutDataTypeStr=Inherit: Inherit via back propagation
  GSOL : Outport
  wires:
  Gain1/1 -> Integrator/1
  Sum/1 -> Max/1, Gain1/1
  FmSOL/1 -> Sum/2
  Gain/1 -> Sum/1
  Integrator/1 -> Gain/1
  Zero/1 -> Max/2
  Max/1 -> GSOL/1

== system nms_sim_2D_cost/CPG-reflex Controller/Golgi tendon organ TA ==
  FTA : Inport
  Gain : Gain  Gain=-1
  Gain1 : Gain  Gain=1/tao_golgi
  Integrator : Integrator  InitialCondition=init_fm
  Max : MinMax  Function=max  Inputs=2
  Sum : Sum
  Zero : Constant  Value=0  OutDataTypeStr=Inherit: Inherit via back propagation
  GTA : Outport
  wires:
  Gain1/1 -> Integrator/1
  Sum/1 -> Max/1, Gain1/1
  FTA/1 -> Sum/2
  Gain/1 -> Sum/1
  Integrator/1 -> Gain/1
  Zero/1 -> Max/2
  Max/1 -> GTA/1

== system nms_sim_2D_cost/CPG-reflex Controller/Golgi tendon organ TA2 ==
  FTA : Inport
  Gain : Gain  Gain=-1
  Gain1 : Gain  Gain=1/tao_golgi
  Integrator : Integrator  InitialCondition=init_fm
  Max : MinMax  Function=max  Inputs=2
  Sum : Sum
  Zero : Constant  Value=0  OutDataTypeStr=Inherit: Inherit via back propagation
  GTA : Outport
  wires:
  Max/1 -> GTA/1
  Zero/1 -> Max/2
  Integrator/1 -> Gain/1
  Gain/1 -> Sum/1
  FTA/1 -> Sum/2
  Sum/1 -> Gain1/1, Max/1
  Gain1/1 -> Integrator/1

== system nms_sim_2D_cost/CPG-reflex Controller/Golgi tendon organ VAS ==
  FmVAS : Inport
  Gain : Gain  Gain=-1
  Gain1 : Gain  Gain=1/tao_golgi
  Integrator : Integrator  InitialCondition=init_fm
  Max : MinMax  Function=max  Inputs=2
  Sum : Sum
  Zero : Constant  Value=0  OutDataTypeStr=Inherit: Inherit via back propagation
  GVAS : Outport
  wires:
  Max/1 -> GVAS/1
  Zero/1 -> Max/2
  Integrator/1 -> Gain/1
  Gain/1 -> Sum/1
  FmVAS/1 -> Sum/2
  Sum/1 -> Gain1/1, Max/1
  Gain1/1 -> Integrator/1

== system nms_sim_2D_cost/CPG-reflex Controller/Golgi tendon organ VAS2 ==
  FmVAS : Inport
  Gain : Gain  Gain=-1
  Gain1 : Gain  Gain=1/tao_golgi
  Integrator : Integrator  InitialCondition=init_fm
  Max : MinMax  Function=max  Inputs=2
  Sum : Sum
  Zero : Constant  Value=0  OutDataTypeStr=Inherit: Inherit via back propagation
  GVAS : Outport
  wires:
  Gain1/1 -> Integrator/1
  Sum/1 -> Max/1, Gain1/1
  FmVAS/1 -> Sum/2
  Gain/1 -> Sum/1
  Integrator/1 -> Gain/1
  Zero/1 -> Max/2
  Max/1 -> GVAS/1

== system nms_sim_2D_cost/CPG-reflex Controller/Muscle Spindle BFSH ==
  note: Lm
  Lce : Inport
  Vce : Inport  Port=2
  Constant2 : Constant
  Constant3 : Constant  Value=0
  Constant4 : Constant
  Gain2 : Gain  Gain=1/tao_spindle
  Gain3 : Gain  Gain=p_BFSH
  Gain4 : Gain  Gain=q_BFSH
  GreaterThan : RelationalOperator  OutDataTypeStr=boolean  RndMeth=Simplest  InputSameDT=off
  Integrator : Integrator  InitialCondition=init_lce
  Saturation : Saturate  UpperLimit=inf  LowerLimit=0
  Saturation1 : Saturate  UpperLimit=inf  LowerLimit=0
  Saturation2 : Saturate  UpperLimit=inf  LowerLimit=0
  Sum4 : Sum  Inputs=|+-
  Sum5 : Sum  Inputs=-++
  Switch : Switch  Criteria=u2 > Threshold  SaturateOnIntegerOverflow=off  InputSameDT=off
  Sm : Outport
  wires:
  Constant2/1 -> Sum4/2
  Saturation/1 -> Gain4/1
  Constant3/1 -> Switch/3
  Constant4/1 -> GreaterThan/2
  GreaterThan/1 -> Switch/2
  Switch/1 -> Sm/1  "Sm"
  Saturation2/1 -> Switch/1
  Gain2/1 -> Integrator/1
  Lce/1 -> Sum4/1, GreaterThan/1  "Lm"
  Saturation1/1 -> Gain3/1
  Gain4/1 -> Sum5/2
  Sum5/1 -> Saturation2/1, Gain2/1
  Integrator/1 -> Sum5/1
  Gain3/1 -> Sum5/3
  Sum4/1 -> Saturation/1
  Vce/1 -> Saturation1/1  "vm"

== system nms_sim_2D_cost/CPG-reflex Controller/Muscle Spindle BFSH2 ==
  note: Lm
  Lce : Inport
  Vce : Inport  Port=2
  Constant2 : Constant
  Constant3 : Constant  Value=0
  Constant4 : Constant
  Gain2 : Gain  Gain=1/tao_spindle
  Gain3 : Gain  Gain=p_BFSH
  Gain4 : Gain  Gain=q_BFSH
  GreaterThan : RelationalOperator  OutDataTypeStr=boolean  RndMeth=Simplest  InputSameDT=off
  Integrator : Integrator  InitialCondition=init_lce
  Saturation : Saturate  UpperLimit=inf  LowerLimit=0
  Saturation1 : Saturate  UpperLimit=inf  LowerLimit=0
  Saturation2 : Saturate  UpperLimit=inf  LowerLimit=0
  Sum4 : Sum  Inputs=|+-
  Sum5 : Sum  Inputs=-++
  Switch : Switch  Criteria=u2 > Threshold  SaturateOnIntegerOverflow=off  InputSameDT=off
  Sm : Outport
  wires:
  Constant2/1 -> Sum4/2
  Saturation/1 -> Gain4/1
  Constant3/1 -> Switch/3
  Constant4/1 -> GreaterThan/2
  GreaterThan/1 -> Switch/2
  Switch/1 -> Sm/1  "Sm"
  Saturation2/1 -> Switch/1
  Gain2/1 -> Integrator/1
  Lce/1 -> Sum4/1, GreaterThan/1  "Lm"
  Saturation1/1 -> Gain3/1
  Gain4/1 -> Sum5/2
  Sum5/1 -> Saturation2/1, Gain2/1
  Integrator/1 -> Sum5/1
  Gain3/1 -> Sum5/3
  Sum4/1 -> Saturation/1
  Vce/1 -> Saturation1/1  "vm"

== system nms_sim_2D_cost/CPG-reflex Controller/Muscle Spindle GAS ==
  note: Lm
  Lce : Inport
  Vce : Inport  Port=2
  Constant2 : Constant
  Constant3 : Constant  Value=0
  Constant4 : Constant
  Gain2 : Gain  Gain=1/tao_spindle
  Gain3 : Gain  Gain=p_GAS
  Gain4 : Gain  Gain=q_GAS
  GreaterThan : RelationalOperator  OutDataTypeStr=boolean  RndMeth=Simplest  InputSameDT=off
  Integrator : Integrator  InitialCondition=init_lce
  Saturation : Saturate  UpperLimit=inf  LowerLimit=0
  Saturation1 : Saturate  UpperLimit=inf  LowerLimit=0
  Saturation2 : Saturate  UpperLimit=inf  LowerLimit=0
  Sum4 : Sum  Inputs=|+-
  Sum5 : Sum  Inputs=-++
  Switch : Switch  Criteria=u2 > Threshold  SaturateOnIntegerOverflow=off  InputSameDT=off
  Sm : Outport
  wires:
  Constant2/1 -> Sum4/2
  Saturation/1 -> Gain4/1
  Constant3/1 -> Switch/3
  Constant4/1 -> GreaterThan/2
  GreaterThan/1 -> Switch/2
  Switch/1 -> Sm/1  "Sm"
  Saturation2/1 -> Switch/1
  Gain2/1 -> Integrator/1
  Lce/1 -> Sum4/1, GreaterThan/1  "Lm"
  Saturation1/1 -> Gain3/1
  Gain4/1 -> Sum5/2
  Sum5/1 -> Saturation2/1, Gain2/1
  Integrator/1 -> Sum5/1
  Gain3/1 -> Sum5/3
  Sum4/1 -> Saturation/1
  Vce/1 -> Saturation1/1  "vm"

== system nms_sim_2D_cost/CPG-reflex Controller/Muscle Spindle GAS2 ==
  note: Lm
  Lce : Inport
  Vce : Inport  Port=2
  Constant2 : Constant
  Constant3 : Constant  Value=0
  Constant4 : Constant
  Gain2 : Gain  Gain=1/tao_spindle
  Gain3 : Gain  Gain=p_GAS
  Gain4 : Gain  Gain=q_GAS
  GreaterThan : RelationalOperator  OutDataTypeStr=boolean  RndMeth=Simplest  InputSameDT=off
  Integrator : Integrator  InitialCondition=init_lce
  Saturation : Saturate  UpperLimit=inf  LowerLimit=0
  Saturation1 : Saturate  UpperLimit=inf  LowerLimit=0
  Saturation2 : Saturate  UpperLimit=inf  LowerLimit=0
  Sum4 : Sum  Inputs=|+-
  Sum5 : Sum  Inputs=-++
  Switch : Switch  Criteria=u2 > Threshold  SaturateOnIntegerOverflow=off  InputSameDT=off
  Sm : Outport
  wires:
  Constant2/1 -> Sum4/2
  Saturation/1 -> Gain4/1
  Constant3/1 -> Switch/3
  Constant4/1 -> GreaterThan/2
  GreaterThan/1 -> Switch/2
  Switch/1 -> Sm/1  "Sm"
  Saturation2/1 -> Switch/1
  Gain2/1 -> Integrator/1
  Lce/1 -> Sum4/1, GreaterThan/1  "Lm"
  Saturation1/1 -> Gain3/1
  Gain4/1 -> Sum5/2
  Sum5/1 -> Saturation2/1, Gain2/1
  Integrator/1 -> Sum5/1
  Gain3/1 -> Sum5/3
  Sum4/1 -> Saturation/1
  Vce/1 -> Saturation1/1  "vm"
